simulink model "1BLDCSpeedControl_EV_Layout_v2"  (R2024b)
settings: Solver=ode23t  StartTime=0.0  StopTime=0.1  FixedStep=Ts  MaxStep=5e-4  RelTol=1e-3  EnableMultiTasking=on
PreLoadFcn:
  | BLDCSpeedControlData;
StartFcn:
  | % [EV_DAQ_V5_HOOK]
  | try; EV_DAQ_Builder_V5('AutoInit'); catch ME__daq; fprintf('[DAQ] Auto-init error: %s\n', ME__daq.message); end
StopFcn:
  | % [EV_DAQ_V5_HOOK]
  | try; EV_DAQ_Builder_V5('PostProcess'); catch ME__daq; fprintf('[DAQ] Post-process error: %s\n', ME__daq.message); end
values from neighbouring files (symbols this model uses):
  m = app.Rows(1:app.N, 1) >= 0.9*t    [EV_BlackBox_App.m]
  N = 0    [EV_BlackBox_App.m]
  p = inputParser    [Create_Simulation.m]    (also in EV_BlackBox_App.m = uipanel(parent, 'Title', title); Run_Simulation_Live.m; Run_Simulation_Log.m)
  s = regexprep(msg, '\s+', ' ')    [EV_BlackBox_App.m]    (also in Run_Simulation_Log.m = T.SOC(isfinite(T.SOC)))
undefined symbols (not defined in the file or in its folder): battery_builder_rtmsupport, cells_parallel, cells_series, DiscIntNeverNeededParam, Emax, Emax_thr, emf_max_ev, gcbh, I_cont, I_peak, Ke_ph, Kii, Kiv, Kiw, Kpi, Kpv, Kpw, load_scale, r_wheel, rpm_ramp, rpm_ref, T_Ifilt, Ts, Tsc, Vdc, Vlim_min, wheel_mass
libraries: nesl_utility x19, fl_lib x13, ee_lib x6, sm_lib x3, eeDiscretePi x2, Batteries2_lib x1, SignalEditorBlockLib x1, eePwmGenerator x1, eeGeneralControl x1
(part 2 of 2)

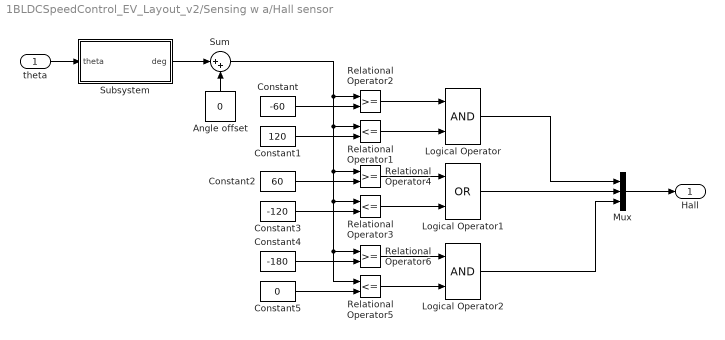
== system 1BLDCSpeedControl_EV_Layout_v2/Sensing w a/Hall sensor ==
  theta : Inport
  Angle offset : Constant  Value=0
  Constant : Constant  Value=-60
  Constant1 : Constant  Value=120
  Constant2 : Constant  Value=60
  Constant3 : Constant  Value=-120
  Constant4 : Constant  Value=-180
  Constant5 : Constant  Value=0
  Logical Operator : Logic  AllPortsSameDT=off  OutDataTypeStr=boolean
  Logical Operator1 : Logic  Operator=OR  AllPortsSameDT=off  OutDataTypeStr=boolean
  Logical Operator2 : Logic  AllPortsSameDT=off  OutDataTypeStr=boolean
  Mux : Mux  Inputs=3
  Relational Operator1 : RelationalOperator  Operator=<=
  Relational Operator2 : RelationalOperator
  Relational Operator3 : RelationalOperator  Operator=<=
  Relational Operator4 : RelationalOperator
  Relational Operator5 : RelationalOperator  Operator=<=
  Relational Operator6 : RelationalOperator
  Subsystem : Subsystem
  Sum : Sum  Inputs=|++
  Hall : Outport  VectorParamsAs1DForOutWhenUnconnected=off
  wires:
  Constant3/1 -> Relational Operator3/2
  Logical Operator2/1 -> Mux/3
  Logical Operator1/1 -> Mux/2
  Logical Operator/1 -> Mux/1
  Relational Operator5/1 -> Logical Operator2/2
  Relational Operator6/1 -> Logical Operator2/1
  Constant4/1 -> Relational Operator6/2
  Constant5/1 -> Relational Operator5/2
  Relational Operator3/1 -> Logical Operator1/2
  Mux/1 -> Hall/1
  Relational Operator2/1 -> Logical Operator/1
  Relational Operator1/1 -> Logical Operator/2
  Constant/1 -> Relational Operator2/2
  Relational Operator4/1 -> Logical Operator1/1
  Constant1/1 -> Relational Operator1/2
  Constant2/1 -> Relational Operator4/2
  theta/1 -> Subsystem/1(theta)
  Subsystem/1(deg) -> Sum/1
  Sum/1 -> Relational Operator1/1, Relational Operator5/1, Relational Operator6/1, Relational Operator3/1, Relational Operator4/1, Relational Operator2/1
  Angle offset/1 -> Sum/2

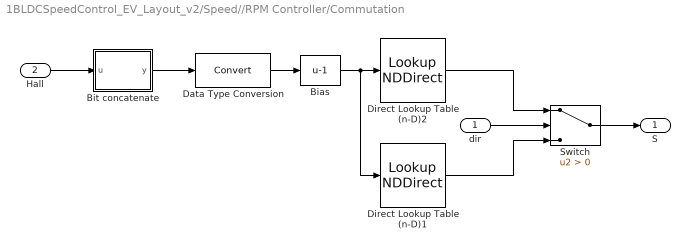
== system 1BLDCSpeedControl_EV_Layout_v2/Speed//RPM Controller/Commutation ==
  dir : Inport
  Hall : Inport  Port=2
  Bias : Bias  Bias=-1  SaturateOnIntegerOverflow=off
  Bit concatenate : Subsystem
  Data Type Conversion : DataTypeConversion  SaturateOnIntegerOverflow=off  RndMeth=Floor
  Direct Lookup Table (n-D)1 : LookupNDDirect  InputsSelectThisObjectFromTable=Vector  Table=[0 1 1 0 0 0;0 0 0 1 1 0;1 0 0 0 1 0;0 1 0 0 0 1;0 0 0 1 0 1;1 0 1 0 0 0]
  Direct Lookup Table (n-D)2 : LookupNDDirect  InputsSelectThisObjectFromTable=Vector  Table=[0 0 0 1 1 0;0 1 1 0 0 0;0 1 0 0 0 1;1 0 0 0 1 0;1 0 1 0 0 0;0 0 0 1 0 1]
  Switch : Switch  Criteria=u2 > Threshold  SaturateOnIntegerOverflow=off  InputSameDT=off
  S : Outport  VectorParamsAs1DForOutWhenUnconnected=off
  wires:
  Hall/1 -> Bit concatenate/1(u)
  Bit concatenate/1(y) -> Data Type Conversion/1
  Data Type Conversion/1 -> Bias/1
  Bias/1 -> Direct Lookup Table (n-D)1/1, Direct Lookup Table (n-D)2/1
  Switch/1 -> S/1
  dir/1 -> Switch/2
  Direct Lookup Table (n-D)2/1 -> Switch/1
  Direct Lookup Table (n-D)1/1 -> Switch/3

== system 1BLDCSpeedControl_EV_Layout_v2/Speed//RPM Controller/PWM ==
  DC : Inport
  Data Type Conversion1 : DataTypeConversion  SaturateOnIntegerOverflow=off  RndMeth=Floor
  Data Type Conversion2 : DataTypeConversion  SaturateOnIntegerOverflow=off  RndMeth=Floor
  Logical Operator : Logic  Operator=NOT  AllPortsSameDT=off  OutDataTypeStr=boolean
  Mux : Mux  Inputs=2
  PWM Generator : eePwmGenerator/PWM Generator  CarrCount=Up  Tper=Tsc  Tdelay=0  Ts=Ts
  Rate Transition4 : RateTransition  OutPortSampleTime=Ts
  G1 : Outport  VectorParamsAs1DForOutWhenUnconnected=off
  wires:
  Mux/1 -> G1/1
  Rate Transition4/1 -> PWM Generator/1
  PWM Generator/1 -> Data Type Conversion2/1, Mux/1
  Data Type Conversion1/1 -> Mux/2
  Logical Operator/1 -> Data Type Conversion1/1
  DC/1 -> Rate Transition4/1
  Data Type Conversion2/1 -> Logical Operator/1

== system 1BLDCSpeedControl_EV_Layout_v2/Speed//RPM Controller/Sign ==
  u : Inport
  Constant2 : Constant
  Constant3 : Constant  Value=-1
  Switch : Switch  SaturateOnIntegerOverflow=off  InputSameDT=off
  y : Outport
  wires:
  Constant3/1 -> Switch/3
  Constant2/1 -> Switch/1
  u/1 -> Switch/2
  Switch/1 -> y/1

== system 1BLDCSpeedControl_EV_Layout_v2/Sensing w a/Hall sensor/Subsystem ==
  theta : Inport
  Trigonometric Function : Trigonometry  Operator=sincos
  Trigonometric Function2 : Trigonometry  Operator=atan2
  mech->elec : Gain  Gain=p
  rad->deg : Gain  Gain=180/pi  SaturateOnIntegerOverflow=on  OutDataTypeStr=Inherit: Same as input  ParamDataTypeStr=Inherit: Same as input
  deg : Outport  VectorParamsAs1DForOutWhenUnconnected=off
  wires:
  Trigonometric Function2/1 -> rad->deg/1
  Trigonometric Function/1 -> Trigonometric Function2/1
  theta/1 -> mech->elec/1
  rad->deg/1 -> deg/1
  Trigonometric Function/2 -> Trigonometric Function2/2
  mech->elec/1 -> Trigonometric Function/1

== system 1BLDCSpeedControl_EV_Layout_v2/Speed//RPM Controller/Commutation/Bit concatenate ==
  u : Inport
  Gain : Gain  Gain=[4 2 1]  Multiplication=Matrix(K*u)
  Sum of Elements : Sum  Inputs=+
  y : Outport  VectorParamsAs1DForOutWhenUnconnected=off
  wires:
  u/1 -> Gain/1
  Gain/1 -> Sum of Elements/1
  Sum of Elements/1 -> y/1
